simulink model "stereo_ibvs_sim_stage1"  (R2025b)
settings: Solver=FixedStepDiscrete  StartTime=0  StopTime=6  FixedStep=cfg.Ts  RelTol=1e-3
PreLoadFcn:
  | %%回调名称	触发时机
  | %PreLoadFcn	打开 slx 模型文件之前执行；适合加载参数、cfg；你这里是空的
  | %PostLoadFcn	模型窗口加载完成之后执行
  | %InitFcn*	点击【运行仿真】，仿真初始化阶段执行（打开模型不会跑，只有启动仿真才运行）
  | %StartFcn	仿真正式开始运行瞬间执行
  | %StopFcn*	仿真停止时执行
  | %CloseFcn*	关闭模型窗口的时候执行
InitFcn:
  | %% 自动定位项目目录、加载视觉伺服配置
  | simFile__    = get_param(bdroot,'FileName');
  | simDir__     = fileparts(simFile__);
  | simulinkDir__= fileparts(simDir__);
  | 
  | coreDir__    = fullfile(simulinkDir__, 'core');
  | configDir__  = fullfile(simulinkDir__, 'config');
  | configFile__ = fullfile(configDir__, 'stereo_ibvs_config.m');
  | 
  | % 加入搜索路径，执行配置脚本
  | addpath(coreDir__);
  | addpath(configDir__);
  | run(configFile__); % 在 InitFcn 局部工作区 逐条运行 stereo_ibvs_config.m 内所有代码,。
  | 
  | %Base 工作区：左侧变量面板（cfg、projectDir、刚体树等）
  | %InitFcn 局部工作区：执行你这段回调代码时，MATLAB 自动开辟的临时独立空间
  | 
  | 
  | % 标记Stage1标定就绪，输出cfg到基础工作区
  | cfg.stage1CalibrationReady = true;
  | assignin('base','cfg', cfg);
  | 
  | % 删除临时局部变量，避免污染base workspace
  | clear simFile__ simDir__ simulinkDir__ coreDir__ configDir__ configFile__
StopFcn:
  | if evalin('base','exist(''cfg'',''var'')==1')
  |     cfg=evalin('base','cfg');
  |     cfg.stage1CalibrationReady=false;
  |     assignin('base','cfg',cfg);
  | end
CloseFcn:
  | %% 如果基础工作区存在cfg，重置Stage1标定就绪标记
  | if evalin('base', 'exist(''cfg'', ''var'') == 1')
  |     cfg = evalin('base', 'cfg');
  |     cfg.stage1CalibrationReady = false;
  |     assignin('base', 'cfg', cfg);
  | end
settings Model: Creator=hlc  LastModifiedBy=harry

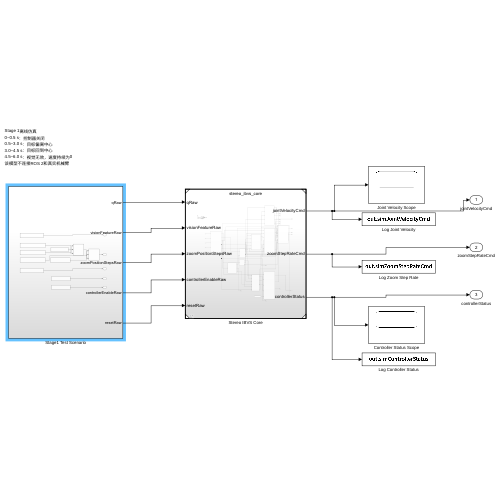
[thumbnail: Simulink's stored preview of the top-level diagram]
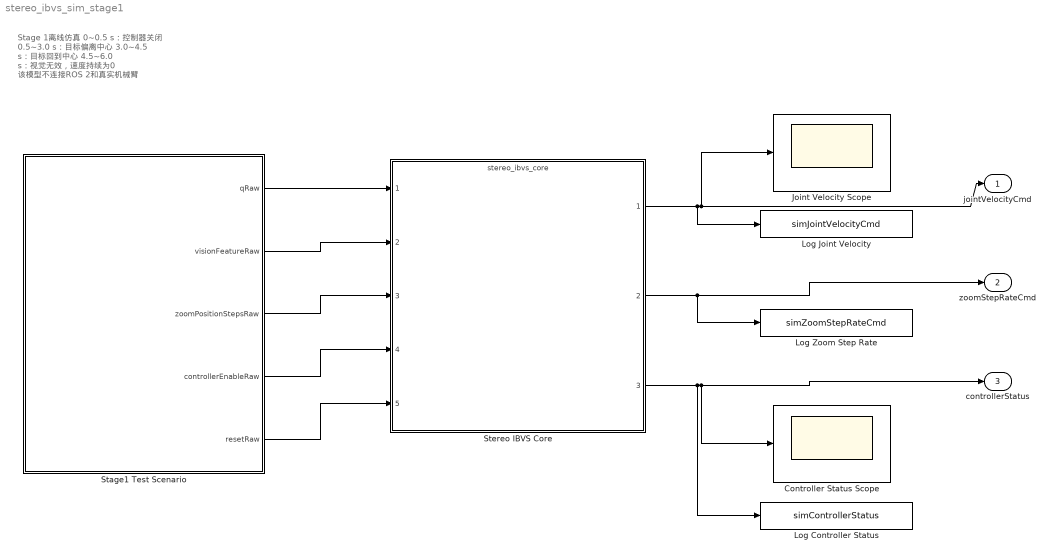
== system stereo_ibvs_sim_stage1 ==
  note: Stage 1离线仿真
      | 0~0.5 s：控制器关闭
      | 0.5~3.0 s：目标偏离中心
      | 3.0~4.5 s：目标回到中心
      | 4.5~6.0 s：视觉无效，速度持续为0
      | 该模型不连接ROS 2和真实机械臂
  Controller Status Scope : Scope
  Joint Velocity Scope : Scope
  Log Controller Status : ToWorkspace  VariableName=simControllerStatus  SaveFormat=Timeseries  SampleTime=-1
  Log Joint Velocity : ToWorkspace  VariableName=simJointVelocityCmd  SaveFormat=Timeseries  SampleTime=-1
  Log Zoom Step Rate : ToWorkspace  VariableName=simZoomStepRateCmd  SaveFormat=Timeseries  SampleTime=-1
  Stage1 Test Scenario : Subsystem
  Stereo IBVS Core : ModelReference  ModelNameDialog=stereo_ibvs_core  SimulationMode=Normal  ModelReferenceVersion=1.49
  jointVelocityCmd : Outport  PortDimensions=[7 1]
  zoomStepRateCmd : Outport  Port=2  PortDimensions=[2 1]
  controllerStatus : Outport  Port=3  PortDimensions=[12 1]
  wires:
  Stage1 Test Scenario/1(qRaw) -> Stereo IBVS Core/1
  Stage1 Test Scenario/2(visionFeatureRaw) -> Stereo IBVS Core/2
  Stage1 Test Scenario/3(zoomPositionStepsRaw) -> Stereo IBVS Core/3
  Stage1 Test Scenario/4(controllerEnableRaw) -> Stereo IBVS Core/4
  Stage1 Test Scenario/5(resetRaw) -> Stereo IBVS Core/5
  Stereo IBVS Core/1 -> jointVelocityCmd/1, Joint Velocity Scope/1, Log Joint Velocity/1
  Stereo IBVS Core/2 -> zoomStepRateCmd/1, Log Zoom Step Rate/1
  Stereo IBVS Core/3 -> controllerStatus/1, Controller Status Scope/1, Log Controller Status/1

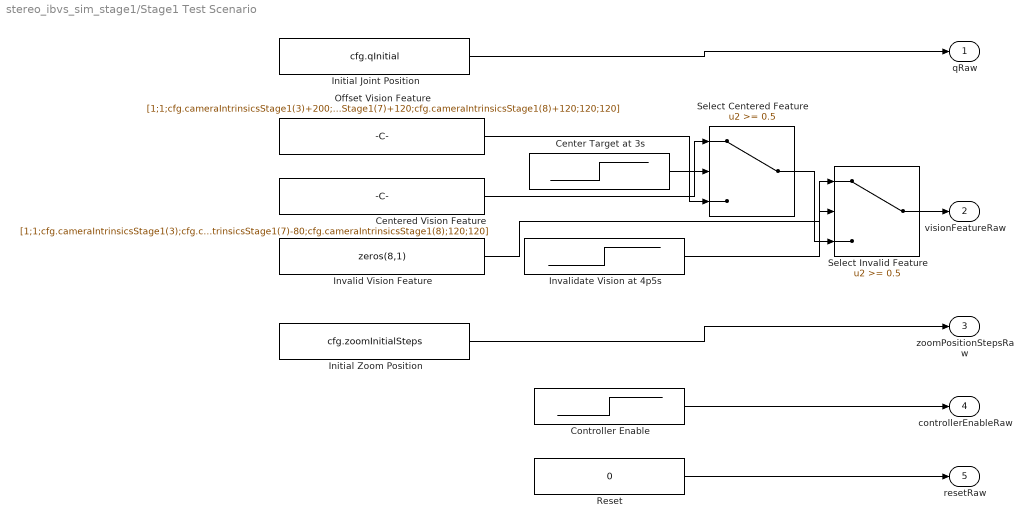
== system stereo_ibvs_sim_stage1/Stage1 Test Scenario ==
  Center Target at 3s : Step  Time=3  SampleTime=cfg.Ts
  Centered Vision Feature : Constant  Value=[1;1;cfg.cameraIntrinsicsStage1(3);cfg.cameraIntrinsicsStage1(4);cfg.cameraIntrinsicsStage1(7)-80;cfg.cameraIntrinsicsStage1(8);120;120]  VectorParams1D=off  OutDataTypeStr=double  SampleTime=cfg.Ts
  Controller Enable : Step  Time=0.5  SampleTime=cfg.Ts
  Initial Joint Position : Constant  Value=cfg.qInitial  VectorParams1D=off  OutDataTypeStr=double  SampleTime=cfg.Ts
  Initial Zoom Position : Constant  Value=cfg.zoomInitialSteps  VectorParams1D=off  OutDataTypeStr=double  SampleTime=cfg.Ts
  Invalid Vision Feature : Constant  Value=zeros(8,1)  VectorParams1D=off  OutDataTypeStr=double  SampleTime=cfg.Ts
  Invalidate Vision at 4p5s : Step  Time=4.5  SampleTime=cfg.Ts
  Offset Vision Feature : Constant  Value=[1;1;cfg.cameraIntrinsicsStage1(3)+200;cfg.cameraIntrinsicsStage1(4)+120;cfg.cameraIntrinsicsStage1(7)+120;cfg.cameraIntrinsicsStage1(8)+120;120;120]  VectorParams1D=off  OutDataTypeStr=double  SampleTime=cfg.Ts
  Reset : Constant  Value=0  OutDataTypeStr=double  SampleTime=cfg.Ts
  Select Centered Feature : Switch  Threshold=0.5  SaturateOnIntegerOverflow=off  InputSameDT=off
  Select Invalid Feature : Switch  Threshold=0.5  SaturateOnIntegerOverflow=off  InputSameDT=off
  qRaw : Outport  PortDimensions=[7 1]
  visionFeatureRaw : Outport  Port=2  PortDimensions=[8 1]
  zoomPositionStepsRaw : Outport  Port=3  PortDimensions=[2 1]
  controllerEnableRaw : Outport  Port=4  PortDimensions=1
  resetRaw : Outport  Port=5  PortDimensions=1
  wires:
  Centered Vision Feature/1 -> Select Centered Feature/1
  Center Target at 3s/1 -> Select Centered Feature/2
  Offset Vision Feature/1 -> Select Centered Feature/3
  Invalid Vision Feature/1 -> Select Invalid Feature/1
  Invalidate Vision at 4p5s/1 -> Select Invalid Feature/2
  Select Centered Feature/1 -> Select Invalid Feature/3
  Initial Joint Position/1 -> qRaw/1
  Select Invalid Feature/1 -> visionFeatureRaw/1
  Initial Zoom Position/1 -> zoomPositionStepsRaw/1
  Controller Enable/1 -> controllerEnableRaw/1
  Reset/1 -> resetRaw/1
